simulink model "ESSSimulation_NCR"  (R2025a)
settings: Solver=VariableStepAuto  StartTime=0.0  StopTime=1800  RelTol=1e-3
undefined symbols (not defined in the file or in its folder): battery_builder_rtmsupport, gcbh
libraries: NCR18650BD_98S45P_Library_lib x14, fl_lib x4, nesl_utility x4, simulink x1, SignalEditorBlockLib x1
(part 2 of 2)

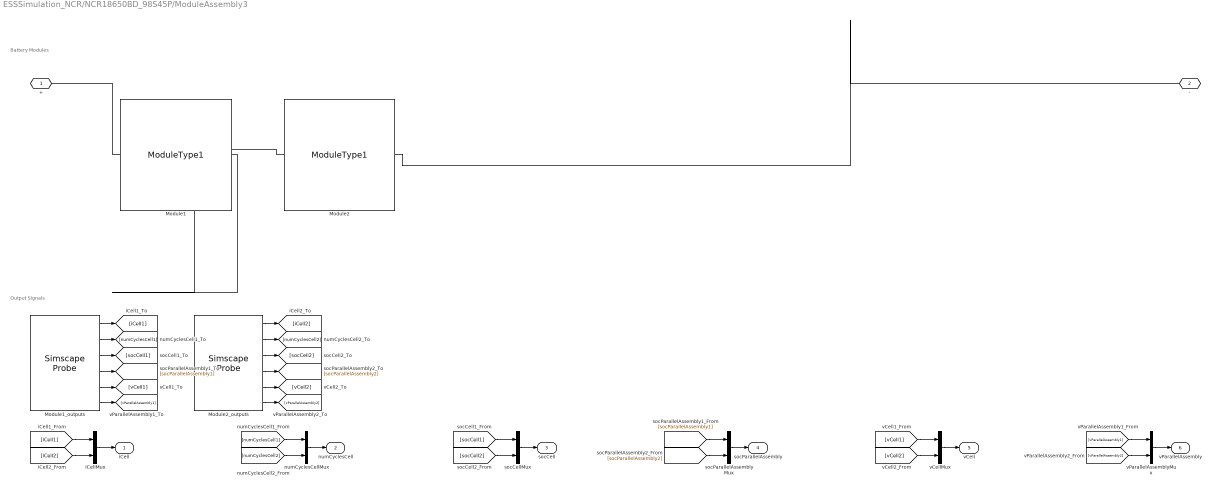
== system ESSSimulation_NCR/NCR18650BD_98S45P/ModuleAssembly3 ==
  note: Battery Modules
  note: Output Signals
  Module1 : NCR18650BD_98S45P_Library_lib/Modules/ModuleType1  SOC_vecCell=[0 0.01 0.02 0.03 0.04 0.05 0.06 0.07 0.08 0.09 0.1 0.11 0.12 0.13 0.14 0.15 0.16 0.17 0.18 0.19 0.2 0.21 0.22 0.23 0.24 0.25 0.26 0.27 0.28 0.29 0.3 0.31 0.32 0.33 0.34 0.35 0.36 0.37 0.38 0.39 0.4 0.41 0.42 0.43 0.44 0.45 0.46 0.47 0.48 0.49 0.5 0.51 0.52 0.53 0.54 0.55 0.56 0.57 0.58 0.59 0.6 0.61 0.62 0.63 0.64 0.65 0.66 0.67 0.68 0.69 0.7 0.71 0.72 0.73 0.74 0.75 0.76 0.77 0.78 0.79 0.8 0.81 0.82 0.83 0.84 0.85 0.86 0.87 0.88 0.89 0.9 0.91 0.92 0.93 0.94 0.95 0.96 0.97 0.98 0.99 1]  V0_vecCell=[2.90003 2.94341 2.98679 3.04987 3.09433 3.12791 3.16031 3.20369 3.23862 3.26689 3.29115 3.31383 3.33202 3.35112 3.36833 3.38413 3.39973 3.41137 3.42149 3.43136 3.44073 3.45027 3.46068 3.47113 3.47814 3.48494 3.49199 3.49905 3.50562 3.51187 3.51861 3.52535 3.53209 3.53818 3.54353 3.54849 3.55353 3.55855 3.56357 3.56831 3.57308 3.57787 3.58264 3.58755 3.5925 3.5985 3.60496 3.61149 3.61805 3.6246 3.63116 3.63855 3.64609 3.65336 3.66064 3.66791 3.67613 3.68522 3.69443 3.70367 3.713 3.72241 3.73154 3.74037 3.7492 3.75786 3.76617 3.77556 3.78485 3.79413 3.8034 3.81149 3.81977 3.82804 3.83631 3.84472 3.85317 3.86155 3.86993 3.87831 3.88686 3.89534 3.90461 3.91454 3.92565 3.93721 3.94924 3.96155 3.97383 3.98598 3.99856 4.01117 4.02361 4.03609 4.04694 4.05695 4.06641 4.07551 4.08514 4.09447 4.10453] V  V_rangeCell=[2.25 Inf] V  R0_vecCell=[0.1741 0.15823 0.14313 0.13285 0.12044 0.10641 0.09605 0.09162 0.08758 0.08349 0.08021 0.07738 0.07487 0.07338 0.07189 0.07117 0.0704 0.06898 0.06755 0.06631 0.06509 0.06388 0.06326 0.06281 0.06182 0.06095 0.06025 0.05955 0.05877 0.05807 0.05761 0.05714 0.05668 0.05611 0.05546 0.0549 0.05439 0.05388 0.05337 0.0528 0.05223 0.05165 0.05106 0.05046 0.04986 0.04945 0.04913 0.04883 0.04854 0.04826 0.04797 0.04782 0.04765 0.0473 0.04695 0.04661 0.04638 0.0463 0.04625 0.04621 0.04624 0.04628 0.04628 0.04623 0.04617 0.04599 0.04573 0.0457 0.04568 0.04565 0.04563 0.04535 0.0451 0.04486 0.04461 0.04446 0.04435 0.04423 0.04411 0.044 0.04372 0.04339 0.04323 0.0432 0.04344 0.04374 0.0441 0.04452 0.04494 0.0454 0.04594 0.0463 0.04649 0.04668 0.04629 0.04541 0.04438 0.04326 0.04154 0.03869 0.03326] Ohm  AHCell=3.153 hr*A  extrapolation_optionCell=simscape.enum.extrapolation.nearest  P=45  S=7  iCell_specify=off  iCell_priority=None  iCell=0 A  iCell_nominal_specify=off  iCell_nominal_value=1  iCell_nominal_unit=A  vCell_specify=off  vCell_priority=None  vCell=0 V  vCell_nominal_specify=off  vCell_nominal_value=1  vCell_nominal_unit=V  socCell_specify=off  socCell_priority=High  socCell=1  socCell_nominal_specify=off  socCell_nominal_value=1  socCell_nominal_unit=1  numCyclesCell_specify=off  numCyclesCell_priority=High  numCyclesCell=0  numCyclesCell_nominal_specify=off  numCyclesCell_nominal_value=1  numCyclesCell_nominal_unit=1  vParallelAssembly_specify=off  vParallelAssembly_priority=None  vParallelAssembly=repmat(0, 7, 1) V  vParallelAssembly_nominal_specify=off  vParallelAssembly_nominal_value=1  vParallelAssembly_nominal_unit=V  socParallelAssembly_specify=off  socParallelAssembly_priority=None  socParallelAssembly=repmat(1, 7, 1)  socParallelAssembly_nominal_specify=off  socParallelAssembly_nominal_value=1  socParallelAssembly_nominal_unit=1
      settings: InternalSimscapePortConfiguration="{\"Bottom\":[{\"id\":\"n\",\"label\":\"-\",\"type\":\"foundation.electrical.electrical\"}],\"Left\":[],\"Right\":[],\"Top\":[{\"id\":\"p\",\"label\":\"+\",\"type\":\"foundation.electrical.electrical\"}]}"
  Module1_outputs : SimscapeProbe  BoundBlock=690  Variables="{\"iCell\":{\"Probing\":\"ON\"},\"numCyclesCell\":{\"Probing\":\"ON\"},\"socCell\":{\"Probing\":\"ON\"},\"socParallelAssembly\":{\"Probing\":\"ON\"},\"vCell\":{\"Probing\":\"ON\"},\"vParallelAssembly\":{\"Probing\":\"ON\"}}"
  Module2 : NCR18650BD_98S45P_Library_lib/Modules/ModuleType1  SOC_vecCell=[0 0.01 0.02 0.03 0.04 0.05 0.06 0.07 0.08 0.09 0.1 0.11 0.12 0.13 0.14 0.15 0.16 0.17 0.18 0.19 0.2 0.21 0.22 0.23 0.24 0.25 0.26 0.27 0.28 0.29 0.3 0.31 0.32 0.33 0.34 0.35 0.36 0.37 0.38 0.39 0.4 0.41 0.42 0.43 0.44 0.45 0.46 0.47 0.48 0.49 0.5 0.51 0.52 0.53 0.54 0.55 0.56 0.57 0.58 0.59 0.6 0.61 0.62 0.63 0.64 0.65 0.66 0.67 0.68 0.69 0.7 0.71 0.72 0.73 0.74 0.75 0.76 0.77 0.78 0.79 0.8 0.81 0.82 0.83 0.84 0.85 0.86 0.87 0.88 0.89 0.9 0.91 0.92 0.93 0.94 0.95 0.96 0.97 0.98 0.99 1]  V0_vecCell=[2.90003 2.94341 2.98679 3.04987 3.09433 3.12791 3.16031 3.20369 3.23862 3.26689 3.29115 3.31383 3.33202 3.35112 3.36833 3.38413 3.39973 3.41137 3.42149 3.43136 3.44073 3.45027 3.46068 3.47113 3.47814 3.48494 3.49199 3.49905 3.50562 3.51187 3.51861 3.52535 3.53209 3.53818 3.54353 3.54849 3.55353 3.55855 3.56357 3.56831 3.57308 3.57787 3.58264 3.58755 3.5925 3.5985 3.60496 3.61149 3.61805 3.6246 3.63116 3.63855 3.64609 3.65336 3.66064 3.66791 3.67613 3.68522 3.69443 3.70367 3.713 3.72241 3.73154 3.74037 3.7492 3.75786 3.76617 3.77556 3.78485 3.79413 3.8034 3.81149 3.81977 3.82804 3.83631 3.84472 3.85317 3.86155 3.86993 3.87831 3.88686 3.89534 3.90461 3.91454 3.92565 3.93721 3.94924 3.96155 3.97383 3.98598 3.99856 4.01117 4.02361 4.03609 4.04694 4.05695 4.06641 4.07551 4.08514 4.09447 4.10453] V  V_rangeCell=[2.25 Inf] V  R0_vecCell=[0.1741 0.15823 0.14313 0.13285 0.12044 0.10641 0.09605 0.09162 0.08758 0.08349 0.08021 0.07738 0.07487 0.07338 0.07189 0.07117 0.0704 0.06898 0.06755 0.06631 0.06509 0.06388 0.06326 0.06281 0.06182 0.06095 0.06025 0.05955 0.05877 0.05807 0.05761 0.05714 0.05668 0.05611 0.05546 0.0549 0.05439 0.05388 0.05337 0.0528 0.05223 0.05165 0.05106 0.05046 0.04986 0.04945 0.04913 0.04883 0.04854 0.04826 0.04797 0.04782 0.04765 0.0473 0.04695 0.04661 0.04638 0.0463 0.04625 0.04621 0.04624 0.04628 0.04628 0.04623 0.04617 0.04599 0.04573 0.0457 0.04568 0.04565 0.04563 0.04535 0.0451 0.04486 0.04461 0.04446 0.04435 0.04423 0.04411 0.044 0.04372 0.04339 0.04323 0.0432 0.04344 0.04374 0.0441 0.04452 0.04494 0.0454 0.04594 0.0463 0.04649 0.04668 0.04629 0.04541 0.04438 0.04326 0.04154 0.03869 0.03326] Ohm  AHCell=3.153 hr*A  extrapolation_optionCell=simscape.enum.extrapolation.nearest  P=45  S=7  iCell_specify=off  iCell_priority=None  iCell=0 A  iCell_nominal_specify=off  iCell_nominal_value=1  iCell_nominal_unit=A  vCell_specify=off  vCell_priority=None  vCell=0 V  vCell_nominal_specify=off  vCell_nominal_value=1  vCell_nominal_unit=V  socCell_specify=off  socCell_priority=High  socCell=1  socCell_nominal_specify=off  socCell_nominal_value=1  socCell_nominal_unit=1  numCyclesCell_specify=off  numCyclesCell_priority=High  numCyclesCell=0  numCyclesCell_nominal_specify=off  numCyclesCell_nominal_value=1  numCyclesCell_nominal_unit=1  vParallelAssembly_specify=off  vParallelAssembly_priority=None  vParallelAssembly=repmat(0, 7, 1) V  vParallelAssembly_nominal_specify=off  vParallelAssembly_nominal_value=1  vParallelAssembly_nominal_unit=V  socParallelAssembly_specify=off  socParallelAssembly_priority=None  socParallelAssembly=repmat(1, 7, 1)  socParallelAssembly_nominal_specify=off  socParallelAssembly_nominal_value=1  socParallelAssembly_nominal_unit=1
      settings: InternalSimscapePortConfiguration="{\"Bottom\":[{\"id\":\"n\",\"label\":\"-\",\"type\":\"foundation.electrical.electrical\"}],\"Left\":[],\"Right\":[],\"Top\":[{\"id\":\"p\",\"label\":\"+\",\"type\":\"foundation.electrical.electrical\"}]}"
  Module2_outputs : SimscapeProbe  BoundBlock=692  Variables="{\"iCell\":{\"Probing\":\"ON\"},\"numCyclesCell\":{\"Probing\":\"ON\"},\"socCell\":{\"Probing\":\"ON\"},\"socParallelAssembly\":{\"Probing\":\"ON\"},\"vCell\":{\"Probing\":\"ON\"},\"vParallelAssembly\":{\"Probing\":\"ON\"}}"
  iCellMux : Mux  Inputs=2
  numCyclesCellMux : Mux  Inputs=2
  socCellMux : Mux  Inputs=2
  socParallelAssemblyMux : Mux  Inputs=2
  vCellMux : Mux  Inputs=2
  vParallelAssemblyMux : Mux  Inputs=2
  + : PMIOPort  Side=Left
  - : PMIOPort  Port=2  Side=Right
  iCell : Outport
  numCyclesCell : Outport  Port=2
  socCell : Outport  Port=3
  socParallelAssembly : Outport  Port=4
  vCell : Outport  Port=5
  vParallelAssembly : Outport  Port=6
  wires:
  Module1_outputs/1 -> [iCell1]
  iCellMux/1 -> iCell/1
  [iCell1] -> iCellMux/1
  Module1_outputs/2 -> [numCyclesCell1]
  numCyclesCellMux/1 -> numCyclesCell/1
  [numCyclesCell1] -> numCyclesCellMux/1
  Module1_outputs/3 -> [socCell1]
  socCellMux/1 -> socCell/1
  [socCell1] -> socCellMux/1
  Module1_outputs/4 -> [socParallelAssembly1]
  socParallelAssemblyMux/1 -> socParallelAssembly/1
  [socParallelAssembly1] -> socParallelAssemblyMux/1
  Module1_outputs/5 -> [vCell1]
  vCellMux/1 -> vCell/1
  [vCell1] -> vCellMux/1
  Module1_outputs/6 -> [vParallelAssembly1]
  vParallelAssemblyMux/1 -> vParallelAssembly/1
  [vParallelAssembly1] -> vParallelAssemblyMux/1
  Module2_outputs/1 -> [iCell2]
  [iCell2] -> iCellMux/2
  Module2_outputs/2 -> [numCyclesCell2]
  [numCyclesCell2] -> numCyclesCellMux/2
  Module2_outputs/3 -> [socCell2]
  [socCell2] -> socCellMux/2
  Module2_outputs/4 -> [socParallelAssembly2]
  [socParallelAssembly2] -> socParallelAssemblyMux/2
  Module2_outputs/5 -> [vCell2]
  [vCell2] -> vCellMux/2
  Module2_outputs/6 -> [vParallelAssembly2]
  [vParallelAssembly2] -> vParallelAssemblyMux/2
  connections:
  Module2/LConn1 -- Module1/RConn1
  Module1/LConn1 -- +/RConn1
  Module2/RConn1 -- -/RConn1

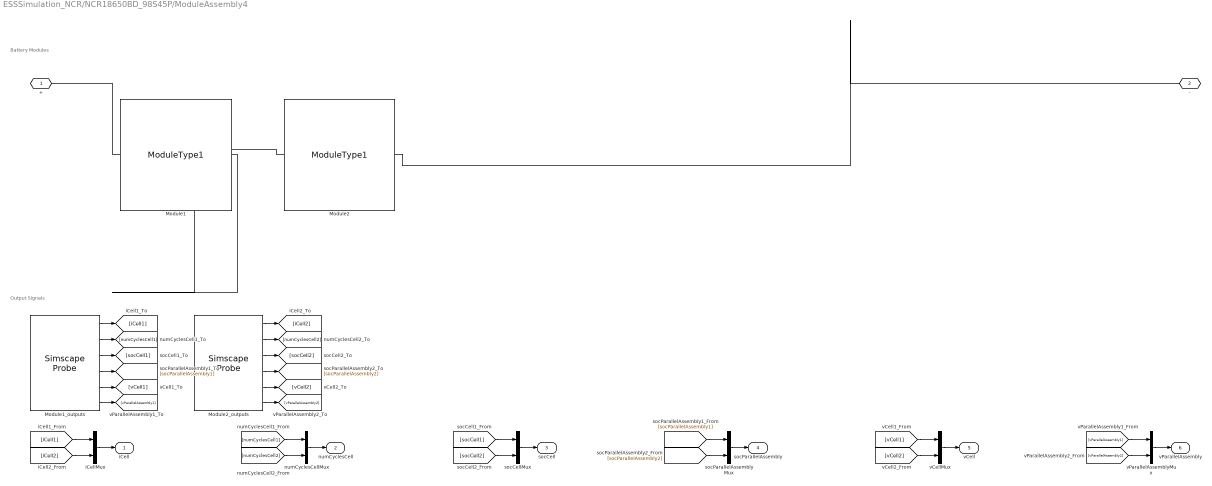
== system ESSSimulation_NCR/NCR18650BD_98S45P/ModuleAssembly4 ==
  note: Battery Modules
  note: Output Signals
  Module1 : NCR18650BD_98S45P_Library_lib/Modules/ModuleType1  SOC_vecCell=[0 0.01 0.02 0.03 0.04 0.05 0.06 0.07 0.08 0.09 0.1 0.11 0.12 0.13 0.14 0.15 0.16 0.17 0.18 0.19 0.2 0.21 0.22 0.23 0.24 0.25 0.26 0.27 0.28 0.29 0.3 0.31 0.32 0.33 0.34 0.35 0.36 0.37 0.38 0.39 0.4 0.41 0.42 0.43 0.44 0.45 0.46 0.47 0.48 0.49 0.5 0.51 0.52 0.53 0.54 0.55 0.56 0.57 0.58 0.59 0.6 0.61 0.62 0.63 0.64 0.65 0.66 0.67 0.68 0.69 0.7 0.71 0.72 0.73 0.74 0.75 0.76 0.77 0.78 0.79 0.8 0.81 0.82 0.83 0.84 0.85 0.86 0.87 0.88 0.89 0.9 0.91 0.92 0.93 0.94 0.95 0.96 0.97 0.98 0.99 1]  V0_vecCell=[2.90003 2.94341 2.98679 3.04987 3.09433 3.12791 3.16031 3.20369 3.23862 3.26689 3.29115 3.31383 3.33202 3.35112 3.36833 3.38413 3.39973 3.41137 3.42149 3.43136 3.44073 3.45027 3.46068 3.47113 3.47814 3.48494 3.49199 3.49905 3.50562 3.51187 3.51861 3.52535 3.53209 3.53818 3.54353 3.54849 3.55353 3.55855 3.56357 3.56831 3.57308 3.57787 3.58264 3.58755 3.5925 3.5985 3.60496 3.61149 3.61805 3.6246 3.63116 3.63855 3.64609 3.65336 3.66064 3.66791 3.67613 3.68522 3.69443 3.70367 3.713 3.72241 3.73154 3.74037 3.7492 3.75786 3.76617 3.77556 3.78485 3.79413 3.8034 3.81149 3.81977 3.82804 3.83631 3.84472 3.85317 3.86155 3.86993 3.87831 3.88686 3.89534 3.90461 3.91454 3.92565 3.93721 3.94924 3.96155 3.97383 3.98598 3.99856 4.01117 4.02361 4.03609 4.04694 4.05695 4.06641 4.07551 4.08514 4.09447 4.10453] V  V_rangeCell=[2.25 Inf] V  R0_vecCell=[0.1741 0.15823 0.14313 0.13285 0.12044 0.10641 0.09605 0.09162 0.08758 0.08349 0.08021 0.07738 0.07487 0.07338 0.07189 0.07117 0.0704 0.06898 0.06755 0.06631 0.06509 0.06388 0.06326 0.06281 0.06182 0.06095 0.06025 0.05955 0.05877 0.05807 0.05761 0.05714 0.05668 0.05611 0.05546 0.0549 0.05439 0.05388 0.05337 0.0528 0.05223 0.05165 0.05106 0.05046 0.04986 0.04945 0.04913 0.04883 0.04854 0.04826 0.04797 0.04782 0.04765 0.0473 0.04695 0.04661 0.04638 0.0463 0.04625 0.04621 0.04624 0.04628 0.04628 0.04623 0.04617 0.04599 0.04573 0.0457 0.04568 0.04565 0.04563 0.04535 0.0451 0.04486 0.04461 0.04446 0.04435 0.04423 0.04411 0.044 0.04372 0.04339 0.04323 0.0432 0.04344 0.04374 0.0441 0.04452 0.04494 0.0454 0.04594 0.0463 0.04649 0.04668 0.04629 0.04541 0.04438 0.04326 0.04154 0.03869 0.03326] Ohm  AHCell=3.153 hr*A  extrapolation_optionCell=simscape.enum.extrapolation.nearest  P=45  S=7  iCell_specify=off  iCell_priority=None  iCell=0 A  iCell_nominal_specify=off  iCell_nominal_value=1  iCell_nominal_unit=A  vCell_specify=off  vCell_priority=None  vCell=0 V  vCell_nominal_specify=off  vCell_nominal_value=1  vCell_nominal_unit=V  socCell_specify=off  socCell_priority=High  socCell=1  socCell_nominal_specify=off  socCell_nominal_value=1  socCell_nominal_unit=1  numCyclesCell_specify=off  numCyclesCell_priority=High  numCyclesCell=0  numCyclesCell_nominal_specify=off  numCyclesCell_nominal_value=1  numCyclesCell_nominal_unit=1  vParallelAssembly_specify=off  vParallelAssembly_priority=None  vParallelAssembly=repmat(0, 7, 1) V  vParallelAssembly_nominal_specify=off  vParallelAssembly_nominal_value=1  vParallelAssembly_nominal_unit=V  socParallelAssembly_specify=off  socParallelAssembly_priority=None  socParallelAssembly=repmat(1, 7, 1)  socParallelAssembly_nominal_specify=off  socParallelAssembly_nominal_value=1  socParallelAssembly_nominal_unit=1
      settings: InternalSimscapePortConfiguration="{\"Bottom\":[{\"id\":\"n\",\"label\":\"-\",\"type\":\"foundation.electrical.electrical\"}],\"Left\":[],\"Right\":[],\"Top\":[{\"id\":\"p\",\"label\":\"+\",\"type\":\"foundation.electrical.electrical\"}]}"
  Module1_outputs : SimscapeProbe  BoundBlock=735  Variables="{\"iCell\":{\"Probing\":\"ON\"},\"numCyclesCell\":{\"Probing\":\"ON\"},\"socCell\":{\"Probing\":\"ON\"},\"socParallelAssembly\":{\"Probing\":\"ON\"},\"vCell\":{\"Probing\":\"ON\"},\"vParallelAssembly\":{\"Probing\":\"ON\"}}"
  Module2 : NCR18650BD_98S45P_Library_lib/Modules/ModuleType1  SOC_vecCell=[0 0.01 0.02 0.03 0.04 0.05 0.06 0.07 0.08 0.09 0.1 0.11 0.12 0.13 0.14 0.15 0.16 0.17 0.18 0.19 0.2 0.21 0.22 0.23 0.24 0.25 0.26 0.27 0.28 0.29 0.3 0.31 0.32 0.33 0.34 0.35 0.36 0.37 0.38 0.39 0.4 0.41 0.42 0.43 0.44 0.45 0.46 0.47 0.48 0.49 0.5 0.51 0.52 0.53 0.54 0.55 0.56 0.57 0.58 0.59 0.6 0.61 0.62 0.63 0.64 0.65 0.66 0.67 0.68 0.69 0.7 0.71 0.72 0.73 0.74 0.75 0.76 0.77 0.78 0.79 0.8 0.81 0.82 0.83 0.84 0.85 0.86 0.87 0.88 0.89 0.9 0.91 0.92 0.93 0.94 0.95 0.96 0.97 0.98 0.99 1]  V0_vecCell=[2.90003 2.94341 2.98679 3.04987 3.09433 3.12791 3.16031 3.20369 3.23862 3.26689 3.29115 3.31383 3.33202 3.35112 3.36833 3.38413 3.39973 3.41137 3.42149 3.43136 3.44073 3.45027 3.46068 3.47113 3.47814 3.48494 3.49199 3.49905 3.50562 3.51187 3.51861 3.52535 3.53209 3.53818 3.54353 3.54849 3.55353 3.55855 3.56357 3.56831 3.57308 3.57787 3.58264 3.58755 3.5925 3.5985 3.60496 3.61149 3.61805 3.6246 3.63116 3.63855 3.64609 3.65336 3.66064 3.66791 3.67613 3.68522 3.69443 3.70367 3.713 3.72241 3.73154 3.74037 3.7492 3.75786 3.76617 3.77556 3.78485 3.79413 3.8034 3.81149 3.81977 3.82804 3.83631 3.84472 3.85317 3.86155 3.86993 3.87831 3.88686 3.89534 3.90461 3.91454 3.92565 3.93721 3.94924 3.96155 3.97383 3.98598 3.99856 4.01117 4.02361 4.03609 4.04694 4.05695 4.06641 4.07551 4.08514 4.09447 4.10453] V  V_rangeCell=[2.25 Inf] V  R0_vecCell=[0.1741 0.15823 0.14313 0.13285 0.12044 0.10641 0.09605 0.09162 0.08758 0.08349 0.08021 0.07738 0.07487 0.07338 0.07189 0.07117 0.0704 0.06898 0.06755 0.06631 0.06509 0.06388 0.06326 0.06281 0.06182 0.06095 0.06025 0.05955 0.05877 0.05807 0.05761 0.05714 0.05668 0.05611 0.05546 0.0549 0.05439 0.05388 0.05337 0.0528 0.05223 0.05165 0.05106 0.05046 0.04986 0.04945 0.04913 0.04883 0.04854 0.04826 0.04797 0.04782 0.04765 0.0473 0.04695 0.04661 0.04638 0.0463 0.04625 0.04621 0.04624 0.04628 0.04628 0.04623 0.04617 0.04599 0.04573 0.0457 0.04568 0.04565 0.04563 0.04535 0.0451 0.04486 0.04461 0.04446 0.04435 0.04423 0.04411 0.044 0.04372 0.04339 0.04323 0.0432 0.04344 0.04374 0.0441 0.04452 0.04494 0.0454 0.04594 0.0463 0.04649 0.04668 0.04629 0.04541 0.04438 0.04326 0.04154 0.03869 0.03326] Ohm  AHCell=3.153 hr*A  extrapolation_optionCell=simscape.enum.extrapolation.nearest  P=45  S=7  iCell_specify=off  iCell_priority=None  iCell=0 A  iCell_nominal_specify=off  iCell_nominal_value=1  iCell_nominal_unit=A  vCell_specify=off  vCell_priority=None  vCell=0 V  vCell_nominal_specify=off  vCell_nominal_value=1  vCell_nominal_unit=V  socCell_specify=off  socCell_priority=High  socCell=1  socCell_nominal_specify=off  socCell_nominal_value=1  socCell_nominal_unit=1  numCyclesCell_specify=off  numCyclesCell_priority=High  numCyclesCell=0  numCyclesCell_nominal_specify=off  numCyclesCell_nominal_value=1  numCyclesCell_nominal_unit=1  vParallelAssembly_specify=off  vParallelAssembly_priority=None  vParallelAssembly=repmat(0, 7, 1) V  vParallelAssembly_nominal_specify=off  vParallelAssembly_nominal_value=1  vParallelAssembly_nominal_unit=V  socParallelAssembly_specify=off  socParallelAssembly_priority=None  socParallelAssembly=repmat(1, 7, 1)  socParallelAssembly_nominal_specify=off  socParallelAssembly_nominal_value=1  socParallelAssembly_nominal_unit=1
      settings: InternalSimscapePortConfiguration="{\"Bottom\":[{\"id\":\"n\",\"label\":\"-\",\"type\":\"foundation.electrical.electrical\"}],\"Left\":[],\"Right\":[],\"Top\":[{\"id\":\"p\",\"label\":\"+\",\"type\":\"foundation.electrical.electrical\"}]}"
  Module2_outputs : SimscapeProbe  BoundBlock=737  Variables="{\"iCell\":{\"Probing\":\"ON\"},\"numCyclesCell\":{\"Probing\":\"ON\"},\"socCell\":{\"Probing\":\"ON\"},\"socParallelAssembly\":{\"Probing\":\"ON\"},\"vCell\":{\"Probing\":\"ON\"},\"vParallelAssembly\":{\"Probing\":\"ON\"}}"
  iCellMux : Mux  Inputs=2
  numCyclesCellMux : Mux  Inputs=2
  socCellMux : Mux  Inputs=2
  socParallelAssemblyMux : Mux  Inputs=2
  vCellMux : Mux  Inputs=2
  vParallelAssemblyMux : Mux  Inputs=2
  + : PMIOPort  Side=Left
  - : PMIOPort  Port=2  Side=Right
  iCell : Outport
  numCyclesCell : Outport  Port=2
  socCell : Outport  Port=3
  socParallelAssembly : Outport  Port=4
  vCell : Outport  Port=5
  vParallelAssembly : Outport  Port=6
  wires:
  Module1_outputs/1 -> [iCell1]
  iCellMux/1 -> iCell/1
  [iCell1] -> iCellMux/1
  Module1_outputs/2 -> [numCyclesCell1]
  numCyclesCellMux/1 -> numCyclesCell/1
  [numCyclesCell1] -> numCyclesCellMux/1
  Module1_outputs/3 -> [socCell1]
  socCellMux/1 -> socCell/1
  [socCell1] -> socCellMux/1
  Module1_outputs/4 -> [socParallelAssembly1]
  socParallelAssemblyMux/1 -> socParallelAssembly/1
  [socParallelAssembly1] -> socParallelAssemblyMux/1
  Module1_outputs/5 -> [vCell1]
  vCellMux/1 -> vCell/1
  [vCell1] -> vCellMux/1
  Module1_outputs/6 -> [vParallelAssembly1]
  vParallelAssemblyMux/1 -> vParallelAssembly/1
  [vParallelAssembly1] -> vParallelAssemblyMux/1
  Module2_outputs/1 -> [iCell2]
  [iCell2] -> iCellMux/2
  Module2_outputs/2 -> [numCyclesCell2]
  [numCyclesCell2] -> numCyclesCellMux/2
  Module2_outputs/3 -> [socCell2]
  [socCell2] -> socCellMux/2
  Module2_outputs/4 -> [socParallelAssembly2]
  [socParallelAssembly2] -> socParallelAssemblyMux/2
  Module2_outputs/5 -> [vCell2]
  [vCell2] -> vCellMux/2
  Module2_outputs/6 -> [vParallelAssembly2]
  [vParallelAssembly2] -> vParallelAssemblyMux/2
  connections:
  Module2/LConn1 -- Module1/RConn1
  Module1/LConn1 -- +/RConn1
  Module2/RConn1 -- -/RConn1

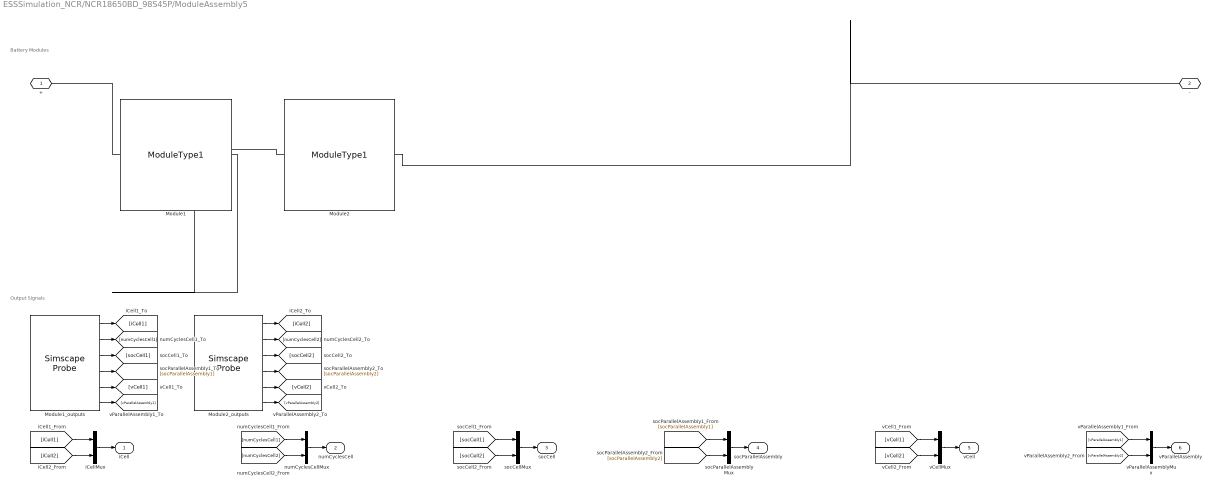
== system ESSSimulation_NCR/NCR18650BD_98S45P/ModuleAssembly5 ==
  note: Battery Modules
  note: Output Signals
  Module1 : NCR18650BD_98S45P_Library_lib/Modules/ModuleType1  SOC_vecCell=[0 0.01 0.02 0.03 0.04 0.05 0.06 0.07 0.08 0.09 0.1 0.11 0.12 0.13 0.14 0.15 0.16 0.17 0.18 0.19 0.2 0.21 0.22 0.23 0.24 0.25 0.26 0.27 0.28 0.29 0.3 0.31 0.32 0.33 0.34 0.35 0.36 0.37 0.38 0.39 0.4 0.41 0.42 0.43 0.44 0.45 0.46 0.47 0.48 0.49 0.5 0.51 0.52 0.53 0.54 0.55 0.56 0.57 0.58 0.59 0.6 0.61 0.62 0.63 0.64 0.65 0.66 0.67 0.68 0.69 0.7 0.71 0.72 0.73 0.74 0.75 0.76 0.77 0.78 0.79 0.8 0.81 0.82 0.83 0.84 0.85 0.86 0.87 0.88 0.89 0.9 0.91 0.92 0.93 0.94 0.95 0.96 0.97 0.98 0.99 1]  V0_vecCell=[2.90003 2.94341 2.98679 3.04987 3.09433 3.12791 3.16031 3.20369 3.23862 3.26689 3.29115 3.31383 3.33202 3.35112 3.36833 3.38413 3.39973 3.41137 3.42149 3.43136 3.44073 3.45027 3.46068 3.47113 3.47814 3.48494 3.49199 3.49905 3.50562 3.51187 3.51861 3.52535 3.53209 3.53818 3.54353 3.54849 3.55353 3.55855 3.56357 3.56831 3.57308 3.57787 3.58264 3.58755 3.5925 3.5985 3.60496 3.61149 3.61805 3.6246 3.63116 3.63855 3.64609 3.65336 3.66064 3.66791 3.67613 3.68522 3.69443 3.70367 3.713 3.72241 3.73154 3.74037 3.7492 3.75786 3.76617 3.77556 3.78485 3.79413 3.8034 3.81149 3.81977 3.82804 3.83631 3.84472 3.85317 3.86155 3.86993 3.87831 3.88686 3.89534 3.90461 3.91454 3.92565 3.93721 3.94924 3.96155 3.97383 3.98598 3.99856 4.01117 4.02361 4.03609 4.04694 4.05695 4.06641 4.07551 4.08514 4.09447 4.10453] V  V_rangeCell=[2.25 Inf] V  R0_vecCell=[0.1741 0.15823 0.14313 0.13285 0.12044 0.10641 0.09605 0.09162 0.08758 0.08349 0.08021 0.07738 0.07487 0.07338 0.07189 0.07117 0.0704 0.06898 0.06755 0.06631 0.06509 0.06388 0.06326 0.06281 0.06182 0.06095 0.06025 0.05955 0.05877 0.05807 0.05761 0.05714 0.05668 0.05611 0.05546 0.0549 0.05439 0.05388 0.05337 0.0528 0.05223 0.05165 0.05106 0.05046 0.04986 0.04945 0.04913 0.04883 0.04854 0.04826 0.04797 0.04782 0.04765 0.0473 0.04695 0.04661 0.04638 0.0463 0.04625 0.04621 0.04624 0.04628 0.04628 0.04623 0.04617 0.04599 0.04573 0.0457 0.04568 0.04565 0.04563 0.04535 0.0451 0.04486 0.04461 0.04446 0.04435 0.04423 0.04411 0.044 0.04372 0.04339 0.04323 0.0432 0.04344 0.04374 0.0441 0.04452 0.04494 0.0454 0.04594 0.0463 0.04649 0.04668 0.04629 0.04541 0.04438 0.04326 0.04154 0.03869 0.03326] Ohm  AHCell=3.153 hr*A  extrapolation_optionCell=simscape.enum.extrapolation.nearest  P=45  S=7  iCell_specify=off  iCell_priority=None  iCell=0 A  iCell_nominal_specify=off  iCell_nominal_value=1  iCell_nominal_unit=A  vCell_specify=off  vCell_priority=None  vCell=0 V  vCell_nominal_specify=off  vCell_nominal_value=1  vCell_nominal_unit=V  socCell_specify=off  socCell_priority=High  socCell=1  socCell_nominal_specify=off  socCell_nominal_value=1  socCell_nominal_unit=1  numCyclesCell_specify=off  numCyclesCell_priority=High  numCyclesCell=0  numCyclesCell_nominal_specify=off  numCyclesCell_nominal_value=1  numCyclesCell_nominal_unit=1  vParallelAssembly_specify=off  vParallelAssembly_priority=None  vParallelAssembly=repmat(0, 7, 1) V  vParallelAssembly_nominal_specify=off  vParallelAssembly_nominal_value=1  vParallelAssembly_nominal_unit=V  socParallelAssembly_specify=off  socParallelAssembly_priority=None  socParallelAssembly=repmat(1, 7, 1)  socParallelAssembly_nominal_specify=off  socParallelAssembly_nominal_value=1  socParallelAssembly_nominal_unit=1
      settings: InternalSimscapePortConfiguration="{\"Bottom\":[{\"id\":\"n\",\"label\":\"-\",\"type\":\"foundation.electrical.electrical\"}],\"Left\":[],\"Right\":[],\"Top\":[{\"id\":\"p\",\"label\":\"+\",\"type\":\"foundation.electrical.electrical\"}]}"
  Module1_outputs : SimscapeProbe  BoundBlock=780  Variables="{\"iCell\":{\"Probing\":\"ON\"},\"numCyclesCell\":{\"Probing\":\"ON\"},\"socCell\":{\"Probing\":\"ON\"},\"socParallelAssembly\":{\"Probing\":\"ON\"},\"vCell\":{\"Probing\":\"ON\"},\"vParallelAssembly\":{\"Probing\":\"ON\"}}"
  Module2 : NCR18650BD_98S45P_Library_lib/Modules/ModuleType1  SOC_vecCell=[0 0.01 0.02 0.03 0.04 0.05 0.06 0.07 0.08 0.09 0.1 0.11 0.12 0.13 0.14 0.15 0.16 0.17 0.18 0.19 0.2 0.21 0.22 0.23 0.24 0.25 0.26 0.27 0.28 0.29 0.3 0.31 0.32 0.33 0.34 0.35 0.36 0.37 0.38 0.39 0.4 0.41 0.42 0.43 0.44 0.45 0.46 0.47 0.48 0.49 0.5 0.51 0.52 0.53 0.54 0.55 0.56 0.57 0.58 0.59 0.6 0.61 0.62 0.63 0.64 0.65 0.66 0.67 0.68 0.69 0.7 0.71 0.72 0.73 0.74 0.75 0.76 0.77 0.78 0.79 0.8 0.81 0.82 0.83 0.84 0.85 0.86 0.87 0.88 0.89 0.9 0.91 0.92 0.93 0.94 0.95 0.96 0.97 0.98 0.99 1]  V0_vecCell=[2.90003 2.94341 2.98679 3.04987 3.09433 3.12791 3.16031 3.20369 3.23862 3.26689 3.29115 3.31383 3.33202 3.35112 3.36833 3.38413 3.39973 3.41137 3.42149 3.43136 3.44073 3.45027 3.46068 3.47113 3.47814 3.48494 3.49199 3.49905 3.50562 3.51187 3.51861 3.52535 3.53209 3.53818 3.54353 3.54849 3.55353 3.55855 3.56357 3.56831 3.57308 3.57787 3.58264 3.58755 3.5925 3.5985 3.60496 3.61149 3.61805 3.6246 3.63116 3.63855 3.64609 3.65336 3.66064 3.66791 3.67613 3.68522 3.69443 3.70367 3.713 3.72241 3.73154 3.74037 3.7492 3.75786 3.76617 3.77556 3.78485 3.79413 3.8034 3.81149 3.81977 3.82804 3.83631 3.84472 3.85317 3.86155 3.86993 3.87831 3.88686 3.89534 3.90461 3.91454 3.92565 3.93721 3.94924 3.96155 3.97383 3.98598 3.99856 4.01117 4.02361 4.03609 4.04694 4.05695 4.06641 4.07551 4.08514 4.09447 4.10453] V  V_rangeCell=[2.25 Inf] V  R0_vecCell=[0.1741 0.15823 0.14313 0.13285 0.12044 0.10641 0.09605 0.09162 0.08758 0.08349 0.08021 0.07738 0.07487 0.07338 0.07189 0.07117 0.0704 0.06898 0.06755 0.06631 0.06509 0.06388 0.06326 0.06281 0.06182 0.06095 0.06025 0.05955 0.05877 0.05807 0.05761 0.05714 0.05668 0.05611 0.05546 0.0549 0.05439 0.05388 0.05337 0.0528 0.05223 0.05165 0.05106 0.05046 0.04986 0.04945 0.04913 0.04883 0.04854 0.04826 0.04797 0.04782 0.04765 0.0473 0.04695 0.04661 0.04638 0.0463 0.04625 0.04621 0.04624 0.04628 0.04628 0.04623 0.04617 0.04599 0.04573 0.0457 0.04568 0.04565 0.04563 0.04535 0.0451 0.04486 0.04461 0.04446 0.04435 0.04423 0.04411 0.044 0.04372 0.04339 0.04323 0.0432 0.04344 0.04374 0.0441 0.04452 0.04494 0.0454 0.04594 0.0463 0.04649 0.04668 0.04629 0.04541 0.04438 0.04326 0.04154 0.03869 0.03326] Ohm  AHCell=3.153 hr*A  extrapolation_optionCell=simscape.enum.extrapolation.nearest  P=45  S=7  iCell_specify=off  iCell_priority=None  iCell=0 A  iCell_nominal_specify=off  iCell_nominal_value=1  iCell_nominal_unit=A  vCell_specify=off  vCell_priority=None  vCell=0 V  vCell_nominal_specify=off  vCell_nominal_value=1  vCell_nominal_unit=V  socCell_specify=off  socCell_priority=High  socCell=1  socCell_nominal_specify=off  socCell_nominal_value=1  socCell_nominal_unit=1  numCyclesCell_specify=off  numCyclesCell_priority=High  numCyclesCell=0  numCyclesCell_nominal_specify=off  numCyclesCell_nominal_value=1  numCyclesCell_nominal_unit=1  vParallelAssembly_specify=off  vParallelAssembly_priority=None  vParallelAssembly=repmat(0, 7, 1) V  vParallelAssembly_nominal_specify=off  vParallelAssembly_nominal_value=1  vParallelAssembly_nominal_unit=V  socParallelAssembly_specify=off  socParallelAssembly_priority=None  socParallelAssembly=repmat(1, 7, 1)  socParallelAssembly_nominal_specify=off  socParallelAssembly_nominal_value=1  socParallelAssembly_nominal_unit=1
      settings: InternalSimscapePortConfiguration="{\"Bottom\":[{\"id\":\"n\",\"label\":\"-\",\"type\":\"foundation.electrical.electrical\"}],\"Left\":[],\"Right\":[],\"Top\":[{\"id\":\"p\",\"label\":\"+\",\"type\":\"foundation.electrical.electrical\"}]}"
  Module2_outputs : SimscapeProbe  BoundBlock=782  Variables="{\"iCell\":{\"Probing\":\"ON\"},\"numCyclesCell\":{\"Probing\":\"ON\"},\"socCell\":{\"Probing\":\"ON\"},\"socParallelAssembly\":{\"Probing\":\"ON\"},\"vCell\":{\"Probing\":\"ON\"},\"vParallelAssembly\":{\"Probing\":\"ON\"}}"
  iCellMux : Mux  Inputs=2
  numCyclesCellMux : Mux  Inputs=2
  socCellMux : Mux  Inputs=2
  socParallelAssemblyMux : Mux  Inputs=2
  vCellMux : Mux  Inputs=2
  vParallelAssemblyMux : Mux  Inputs=2
  + : PMIOPort  Side=Left
  - : PMIOPort  Port=2  Side=Right
  iCell : Outport
  numCyclesCell : Outport  Port=2
  socCell : Outport  Port=3
  socParallelAssembly : Outport  Port=4
  vCell : Outport  Port=5
  vParallelAssembly : Outport  Port=6
  wires:
  Module1_outputs/1 -> [iCell1]
  iCellMux/1 -> iCell/1
  [iCell1] -> iCellMux/1
  Module1_outputs/2 -> [numCyclesCell1]
  numCyclesCellMux/1 -> numCyclesCell/1
  [numCyclesCell1] -> numCyclesCellMux/1
  Module1_outputs/3 -> [socCell1]
  socCellMux/1 -> socCell/1
  [socCell1] -> socCellMux/1
  Module1_outputs/4 -> [socParallelAssembly1]
  socParallelAssemblyMux/1 -> socParallelAssembly/1
  [socParallelAssembly1] -> socParallelAssemblyMux/1
  Module1_outputs/5 -> [vCell1]
  vCellMux/1 -> vCell/1
  [vCell1] -> vCellMux/1
  Module1_outputs/6 -> [vParallelAssembly1]
  vParallelAssemblyMux/1 -> vParallelAssembly/1
  [vParallelAssembly1] -> vParallelAssemblyMux/1
  Module2_outputs/1 -> [iCell2]
  [iCell2] -> iCellMux/2
  Module2_outputs/2 -> [numCyclesCell2]
  [numCyclesCell2] -> numCyclesCellMux/2
  Module2_outputs/3 -> [socCell2]
  [socCell2] -> socCellMux/2
  Module2_outputs/4 -> [socParallelAssembly2]
  [socParallelAssembly2] -> socParallelAssemblyMux/2
  Module2_outputs/5 -> [vCell2]
  [vCell2] -> vCellMux/2
  Module2_outputs/6 -> [vParallelAssembly2]
  [vParallelAssembly2] -> vParallelAssemblyMux/2
  connections:
  Module2/LConn1 -- Module1/RConn1
  Module1/LConn1 -- +/RConn1
  Module2/RConn1 -- -/RConn1

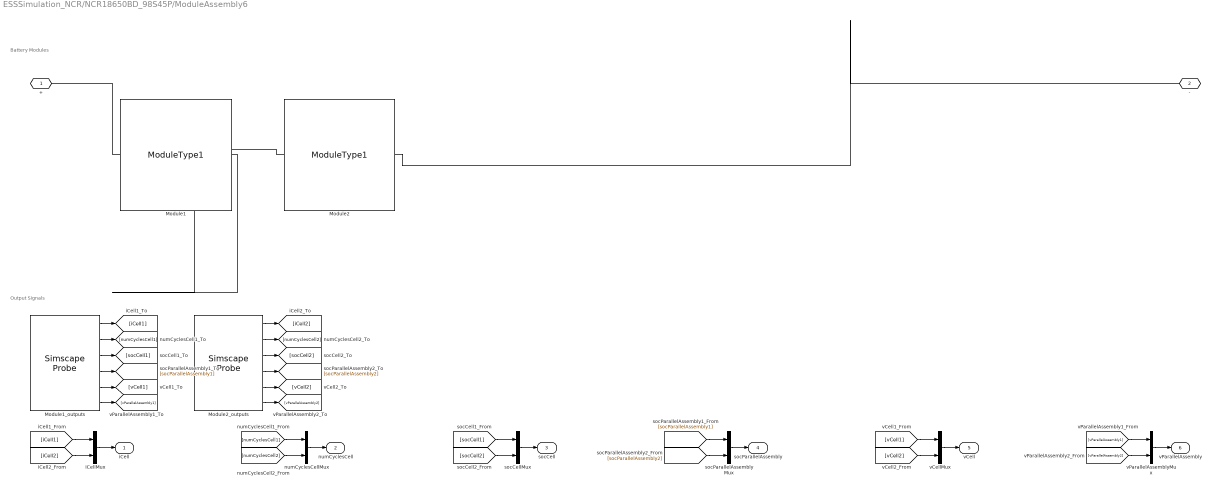
== system ESSSimulation_NCR/NCR18650BD_98S45P/ModuleAssembly6 ==
  note: Battery Modules
  note: Output Signals
  Module1 : NCR18650BD_98S45P_Library_lib/Modules/ModuleType1  SOC_vecCell=[0 0.01 0.02 0.03 0.04 0.05 0.06 0.07 0.08 0.09 0.1 0.11 0.12 0.13 0.14 0.15 0.16 0.17 0.18 0.19 0.2 0.21 0.22 0.23 0.24 0.25 0.26 0.27 0.28 0.29 0.3 0.31 0.32 0.33 0.34 0.35 0.36 0.37 0.38 0.39 0.4 0.41 0.42 0.43 0.44 0.45 0.46 0.47 0.48 0.49 0.5 0.51 0.52 0.53 0.54 0.55 0.56 0.57 0.58 0.59 0.6 0.61 0.62 0.63 0.64 0.65 0.66 0.67 0.68 0.69 0.7 0.71 0.72 0.73 0.74 0.75 0.76 0.77 0.78 0.79 0.8 0.81 0.82 0.83 0.84 0.85 0.86 0.87 0.88 0.89 0.9 0.91 0.92 0.93 0.94 0.95 0.96 0.97 0.98 0.99 1]  V0_vecCell=[2.90003 2.94341 2.98679 3.04987 3.09433 3.12791 3.16031 3.20369 3.23862 3.26689 3.29115 3.31383 3.33202 3.35112 3.36833 3.38413 3.39973 3.41137 3.42149 3.43136 3.44073 3.45027 3.46068 3.47113 3.47814 3.48494 3.49199 3.49905 3.50562 3.51187 3.51861 3.52535 3.53209 3.53818 3.54353 3.54849 3.55353 3.55855 3.56357 3.56831 3.57308 3.57787 3.58264 3.58755 3.5925 3.5985 3.60496 3.61149 3.61805 3.6246 3.63116 3.63855 3.64609 3.65336 3.66064 3.66791 3.67613 3.68522 3.69443 3.70367 3.713 3.72241 3.73154 3.74037 3.7492 3.75786 3.76617 3.77556 3.78485 3.79413 3.8034 3.81149 3.81977 3.82804 3.83631 3.84472 3.85317 3.86155 3.86993 3.87831 3.88686 3.89534 3.90461 3.91454 3.92565 3.93721 3.94924 3.96155 3.97383 3.98598 3.99856 4.01117 4.02361 4.03609 4.04694 4.05695 4.06641 4.07551 4.08514 4.09447 4.10453] V  V_rangeCell=[2.25 Inf] V  R0_vecCell=[0.1741 0.15823 0.14313 0.13285 0.12044 0.10641 0.09605 0.09162 0.08758 0.08349 0.08021 0.07738 0.07487 0.07338 0.07189 0.07117 0.0704 0.06898 0.06755 0.06631 0.06509 0.06388 0.06326 0.06281 0.06182 0.06095 0.06025 0.05955 0.05877 0.05807 0.05761 0.05714 0.05668 0.05611 0.05546 0.0549 0.05439 0.05388 0.05337 0.0528 0.05223 0.05165 0.05106 0.05046 0.04986 0.04945 0.04913 0.04883 0.04854 0.04826 0.04797 0.04782 0.04765 0.0473 0.04695 0.04661 0.04638 0.0463 0.04625 0.04621 0.04624 0.04628 0.04628 0.04623 0.04617 0.04599 0.04573 0.0457 0.04568 0.04565 0.04563 0.04535 0.0451 0.04486 0.04461 0.04446 0.04435 0.04423 0.04411 0.044 0.04372 0.04339 0.04323 0.0432 0.04344 0.04374 0.0441 0.04452 0.04494 0.0454 0.04594 0.0463 0.04649 0.04668 0.04629 0.04541 0.04438 0.04326 0.04154 0.03869 0.03326] Ohm  AHCell=3.153 hr*A  extrapolation_optionCell=simscape.enum.extrapolation.nearest  P=45  S=7  iCell_specify=off  iCell_priority=None  iCell=0 A  iCell_nominal_specify=off  iCell_nominal_value=1  iCell_nominal_unit=A  vCell_specify=off  vCell_priority=None  vCell=0 V  vCell_nominal_specify=off  vCell_nominal_value=1  vCell_nominal_unit=V  socCell_specify=off  socCell_priority=High  socCell=1  socCell_nominal_specify=off  socCell_nominal_value=1  socCell_nominal_unit=1  numCyclesCell_specify=off  numCyclesCell_priority=High  numCyclesCell=0  numCyclesCell_nominal_specify=off  numCyclesCell_nominal_value=1  numCyclesCell_nominal_unit=1  vParallelAssembly_specify=off  vParallelAssembly_priority=None  vParallelAssembly=repmat(0, 7, 1) V  vParallelAssembly_nominal_specify=off  vParallelAssembly_nominal_value=1  vParallelAssembly_nominal_unit=V  socParallelAssembly_specify=off  socParallelAssembly_priority=None  socParallelAssembly=repmat(1, 7, 1)  socParallelAssembly_nominal_specify=off  socParallelAssembly_nominal_value=1  socParallelAssembly_nominal_unit=1
      settings: InternalSimscapePortConfiguration="{\"Bottom\":[{\"id\":\"n\",\"label\":\"-\",\"type\":\"foundation.electrical.electrical\"}],\"Left\":[],\"Right\":[],\"Top\":[{\"id\":\"p\",\"label\":\"+\",\"type\":\"foundation.electrical.electrical\"}]}"
  Module1_outputs : SimscapeProbe  BoundBlock=825  Variables="{\"iCell\":{\"Probing\":\"ON\"},\"numCyclesCell\":{\"Probing\":\"ON\"},\"socCell\":{\"Probing\":\"ON\"},\"socParallelAssembly\":{\"Probing\":\"ON\"},\"vCell\":{\"Probing\":\"ON\"},\"vParallelAssembly\":{\"Probing\":\"ON\"}}"
  Module2 : NCR18650BD_98S45P_Library_lib/Modules/ModuleType1  SOC_vecCell=[0 0.01 0.02 0.03 0.04 0.05 0.06 0.07 0.08 0.09 0.1 0.11 0.12 0.13 0.14 0.15 0.16 0.17 0.18 0.19 0.2 0.21 0.22 0.23 0.24 0.25 0.26 0.27 0.28 0.29 0.3 0.31 0.32 0.33 0.34 0.35 0.36 0.37 0.38 0.39 0.4 0.41 0.42 0.43 0.44 0.45 0.46 0.47 0.48 0.49 0.5 0.51 0.52 0.53 0.54 0.55 0.56 0.57 0.58 0.59 0.6 0.61 0.62 0.63 0.64 0.65 0.66 0.67 0.68 0.69 0.7 0.71 0.72 0.73 0.74 0.75 0.76 0.77 0.78 0.79 0.8 0.81 0.82 0.83 0.84 0.85 0.86 0.87 0.88 0.89 0.9 0.91 0.92 0.93 0.94 0.95 0.96 0.97 0.98 0.99 1]  V0_vecCell=[2.90003 2.94341 2.98679 3.04987 3.09433 3.12791 3.16031 3.20369 3.23862 3.26689 3.29115 3.31383 3.33202 3.35112 3.36833 3.38413 3.39973 3.41137 3.42149 3.43136 3.44073 3.45027 3.46068 3.47113 3.47814 3.48494 3.49199 3.49905 3.50562 3.51187 3.51861 3.52535 3.53209 3.53818 3.54353 3.54849 3.55353 3.55855 3.56357 3.56831 3.57308 3.57787 3.58264 3.58755 3.5925 3.5985 3.60496 3.61149 3.61805 3.6246 3.63116 3.63855 3.64609 3.65336 3.66064 3.66791 3.67613 3.68522 3.69443 3.70367 3.713 3.72241 3.73154 3.74037 3.7492 3.75786 3.76617 3.77556 3.78485 3.79413 3.8034 3.81149 3.81977 3.82804 3.83631 3.84472 3.85317 3.86155 3.86993 3.87831 3.88686 3.89534 3.90461 3.91454 3.92565 3.93721 3.94924 3.96155 3.97383 3.98598 3.99856 4.01117 4.02361 4.03609 4.04694 4.05695 4.06641 4.07551 4.08514 4.09447 4.10453] V  V_rangeCell=[2.25 Inf] V  R0_vecCell=[0.1741 0.15823 0.14313 0.13285 0.12044 0.10641 0.09605 0.09162 0.08758 0.08349 0.08021 0.07738 0.07487 0.07338 0.07189 0.07117 0.0704 0.06898 0.06755 0.06631 0.06509 0.06388 0.06326 0.06281 0.06182 0.06095 0.06025 0.05955 0.05877 0.05807 0.05761 0.05714 0.05668 0.05611 0.05546 0.0549 0.05439 0.05388 0.05337 0.0528 0.05223 0.05165 0.05106 0.05046 0.04986 0.04945 0.04913 0.04883 0.04854 0.04826 0.04797 0.04782 0.04765 0.0473 0.04695 0.04661 0.04638 0.0463 0.04625 0.04621 0.04624 0.04628 0.04628 0.04623 0.04617 0.04599 0.04573 0.0457 0.04568 0.04565 0.04563 0.04535 0.0451 0.04486 0.04461 0.04446 0.04435 0.04423 0.04411 0.044 0.04372 0.04339 0.04323 0.0432 0.04344 0.04374 0.0441 0.04452 0.04494 0.0454 0.04594 0.0463 0.04649 0.04668 0.04629 0.04541 0.04438 0.04326 0.04154 0.03869 0.03326] Ohm  AHCell=3.153 hr*A  extrapolation_optionCell=simscape.enum.extrapolation.nearest  P=45  S=7  iCell_specify=off  iCell_priority=None  iCell=0 A  iCell_nominal_specify=off  iCell_nominal_value=1  iCell_nominal_unit=A  vCell_specify=off  vCell_priority=None  vCell=0 V  vCell_nominal_specify=off  vCell_nominal_value=1  vCell_nominal_unit=V  socCell_specify=off  socCell_priority=High  socCell=1  socCell_nominal_specify=off  socCell_nominal_value=1  socCell_nominal_unit=1  numCyclesCell_specify=off  numCyclesCell_priority=High  numCyclesCell=0  numCyclesCell_nominal_specify=off  numCyclesCell_nominal_value=1  numCyclesCell_nominal_unit=1  vParallelAssembly_specify=off  vParallelAssembly_priority=None  vParallelAssembly=repmat(0, 7, 1) V  vParallelAssembly_nominal_specify=off  vParallelAssembly_nominal_value=1  vParallelAssembly_nominal_unit=V  socParallelAssembly_specify=off  socParallelAssembly_priority=None  socParallelAssembly=repmat(1, 7, 1)  socParallelAssembly_nominal_specify=off  socParallelAssembly_nominal_value=1  socParallelAssembly_nominal_unit=1
      settings: InternalSimscapePortConfiguration="{\"Bottom\":[{\"id\":\"n\",\"label\":\"-\",\"type\":\"foundation.electrical.electrical\"}],\"Left\":[],\"Right\":[],\"Top\":[{\"id\":\"p\",\"label\":\"+\",\"type\":\"foundation.electrical.electrical\"}]}"
  Module2_outputs : SimscapeProbe  BoundBlock=827  Variables="{\"iCell\":{\"Probing\":\"ON\"},\"numCyclesCell\":{\"Probing\":\"ON\"},\"socCell\":{\"Probing\":\"ON\"},\"socParallelAssembly\":{\"Probing\":\"ON\"},\"vCell\":{\"Probing\":\"ON\"},\"vParallelAssembly\":{\"Probing\":\"ON\"}}"
  iCellMux : Mux  Inputs=2
  numCyclesCellMux : Mux  Inputs=2
  socCellMux : Mux  Inputs=2
  socParallelAssemblyMux : Mux  Inputs=2
  vCellMux : Mux  Inputs=2
  vParallelAssemblyMux : Mux  Inputs=2
  + : PMIOPort  Side=Left
  - : PMIOPort  Port=2  Side=Right
  iCell : Outport
  numCyclesCell : Outport  Port=2
  socCell : Outport  Port=3
  socParallelAssembly : Outport  Port=4
  vCell : Outport  Port=5
  vParallelAssembly : Outport  Port=6
  wires:
  Module1_outputs/1 -> [iCell1]
  iCellMux/1 -> iCell/1
  [iCell1] -> iCellMux/1
  Module1_outputs/2 -> [numCyclesCell1]
  numCyclesCellMux/1 -> numCyclesCell/1
  [numCyclesCell1] -> numCyclesCellMux/1
  Module1_outputs/3 -> [socCell1]
  socCellMux/1 -> socCell/1
  [socCell1] -> socCellMux/1
  Module1_outputs/4 -> [socParallelAssembly1]
  socParallelAssemblyMux/1 -> socParallelAssembly/1
  [socParallelAssembly1] -> socParallelAssemblyMux/1
  Module1_outputs/5 -> [vCell1]
  vCellMux/1 -> vCell/1
  [vCell1] -> vCellMux/1
  Module1_outputs/6 -> [vParallelAssembly1]
  vParallelAssemblyMux/1 -> vParallelAssembly/1
  [vParallelAssembly1] -> vParallelAssemblyMux/1
  Module2_outputs/1 -> [iCell2]
  [iCell2] -> iCellMux/2
  Module2_outputs/2 -> [numCyclesCell2]
  [numCyclesCell2] -> numCyclesCellMux/2
  Module2_outputs/3 -> [socCell2]
  [socCell2] -> socCellMux/2
  Module2_outputs/4 -> [socParallelAssembly2]
  [socParallelAssembly2] -> socParallelAssemblyMux/2
  Module2_outputs/5 -> [vCell2]
  [vCell2] -> vCellMux/2
  Module2_outputs/6 -> [vParallelAssembly2]
  [vParallelAssembly2] -> vParallelAssemblyMux/2
  connections:
  Module2/LConn1 -- Module1/RConn1
  Module1/LConn1 -- +/RConn1
  Module2/RConn1 -- -/RConn1

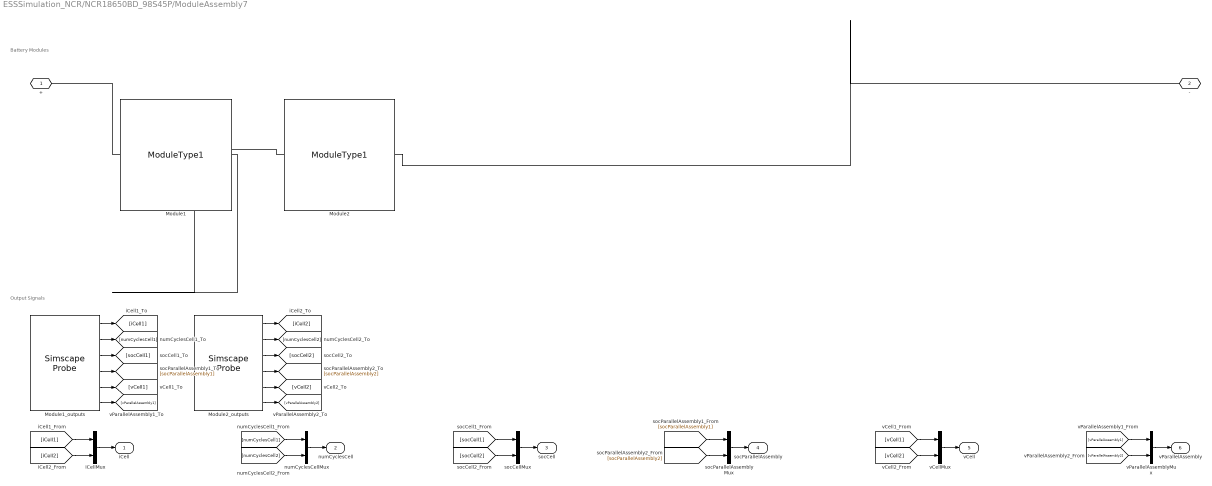
== system ESSSimulation_NCR/NCR18650BD_98S45P/ModuleAssembly7 ==
  note: Battery Modules
  note: Output Signals
  Module1 : NCR18650BD_98S45P_Library_lib/Modules/ModuleType1  SOC_vecCell=[0 0.01 0.02 0.03 0.04 0.05 0.06 0.07 0.08 0.09 0.1 0.11 0.12 0.13 0.14 0.15 0.16 0.17 0.18 0.19 0.2 0.21 0.22 0.23 0.24 0.25 0.26 0.27 0.28 0.29 0.3 0.31 0.32 0.33 0.34 0.35 0.36 0.37 0.38 0.39 0.4 0.41 0.42 0.43 0.44 0.45 0.46 0.47 0.48 0.49 0.5 0.51 0.52 0.53 0.54 0.55 0.56 0.57 0.58 0.59 0.6 0.61 0.62 0.63 0.64 0.65 0.66 0.67 0.68 0.69 0.7 0.71 0.72 0.73 0.74 0.75 0.76 0.77 0.78 0.79 0.8 0.81 0.82 0.83 0.84 0.85 0.86 0.87 0.88 0.89 0.9 0.91 0.92 0.93 0.94 0.95 0.96 0.97 0.98 0.99 1]  V0_vecCell=[2.90003 2.94341 2.98679 3.04987 3.09433 3.12791 3.16031 3.20369 3.23862 3.26689 3.29115 3.31383 3.33202 3.35112 3.36833 3.38413 3.39973 3.41137 3.42149 3.43136 3.44073 3.45027 3.46068 3.47113 3.47814 3.48494 3.49199 3.49905 3.50562 3.51187 3.51861 3.52535 3.53209 3.53818 3.54353 3.54849 3.55353 3.55855 3.56357 3.56831 3.57308 3.57787 3.58264 3.58755 3.5925 3.5985 3.60496 3.61149 3.61805 3.6246 3.63116 3.63855 3.64609 3.65336 3.66064 3.66791 3.67613 3.68522 3.69443 3.70367 3.713 3.72241 3.73154 3.74037 3.7492 3.75786 3.76617 3.77556 3.78485 3.79413 3.8034 3.81149 3.81977 3.82804 3.83631 3.84472 3.85317 3.86155 3.86993 3.87831 3.88686 3.89534 3.90461 3.91454 3.92565 3.93721 3.94924 3.96155 3.97383 3.98598 3.99856 4.01117 4.02361 4.03609 4.04694 4.05695 4.06641 4.07551 4.08514 4.09447 4.10453] V  V_rangeCell=[2.25 Inf] V  R0_vecCell=[0.1741 0.15823 0.14313 0.13285 0.12044 0.10641 0.09605 0.09162 0.08758 0.08349 0.08021 0.07738 0.07487 0.07338 0.07189 0.07117 0.0704 0.06898 0.06755 0.06631 0.06509 0.06388 0.06326 0.06281 0.06182 0.06095 0.06025 0.05955 0.05877 0.05807 0.05761 0.05714 0.05668 0.05611 0.05546 0.0549 0.05439 0.05388 0.05337 0.0528 0.05223 0.05165 0.05106 0.05046 0.04986 0.04945 0.04913 0.04883 0.04854 0.04826 0.04797 0.04782 0.04765 0.0473 0.04695 0.04661 0.04638 0.0463 0.04625 0.04621 0.04624 0.04628 0.04628 0.04623 0.04617 0.04599 0.04573 0.0457 0.04568 0.04565 0.04563 0.04535 0.0451 0.04486 0.04461 0.04446 0.04435 0.04423 0.04411 0.044 0.04372 0.04339 0.04323 0.0432 0.04344 0.04374 0.0441 0.04452 0.04494 0.0454 0.04594 0.0463 0.04649 0.04668 0.04629 0.04541 0.04438 0.04326 0.04154 0.03869 0.03326] Ohm  AHCell=3.153 hr*A  extrapolation_optionCell=simscape.enum.extrapolation.nearest  P=45  S=7  iCell_specify=off  iCell_priority=None  iCell=0 A  iCell_nominal_specify=off  iCell_nominal_value=1  iCell_nominal_unit=A  vCell_specify=off  vCell_priority=None  vCell=0 V  vCell_nominal_specify=off  vCell_nominal_value=1  vCell_nominal_unit=V  socCell_specify=off  socCell_priority=High  socCell=1  socCell_nominal_specify=off  socCell_nominal_value=1  socCell_nominal_unit=1  numCyclesCell_specify=off  numCyclesCell_priority=High  numCyclesCell=0  numCyclesCell_nominal_specify=off  numCyclesCell_nominal_value=1  numCyclesCell_nominal_unit=1  vParallelAssembly_specify=off  vParallelAssembly_priority=None  vParallelAssembly=repmat(0, 7, 1) V  vParallelAssembly_nominal_specify=off  vParallelAssembly_nominal_value=1  vParallelAssembly_nominal_unit=V  socParallelAssembly_specify=off  socParallelAssembly_priority=None  socParallelAssembly=repmat(1, 7, 1)  socParallelAssembly_nominal_specify=off  socParallelAssembly_nominal_value=1  socParallelAssembly_nominal_unit=1
      settings: InternalSimscapePortConfiguration="{\"Bottom\":[{\"id\":\"n\",\"label\":\"-\",\"type\":\"foundation.electrical.electrical\"}],\"Left\":[],\"Right\":[],\"Top\":[{\"id\":\"p\",\"label\":\"+\",\"type\":\"foundation.electrical.electrical\"}]}"
  Module1_outputs : SimscapeProbe  BoundBlock=870  Variables="{\"iCell\":{\"Probing\":\"ON\"},\"numCyclesCell\":{\"Probing\":\"ON\"},\"socCell\":{\"Probing\":\"ON\"},\"socParallelAssembly\":{\"Probing\":\"ON\"},\"vCell\":{\"Probing\":\"ON\"},\"vParallelAssembly\":{\"Probing\":\"ON\"}}"
  Module2 : NCR18650BD_98S45P_Library_lib/Modules/ModuleType1  SOC_vecCell=[0 0.01 0.02 0.03 0.04 0.05 0.06 0.07 0.08 0.09 0.1 0.11 0.12 0.13 0.14 0.15 0.16 0.17 0.18 0.19 0.2 0.21 0.22 0.23 0.24 0.25 0.26 0.27 0.28 0.29 0.3 0.31 0.32 0.33 0.34 0.35 0.36 0.37 0.38 0.39 0.4 0.41 0.42 0.43 0.44 0.45 0.46 0.47 0.48 0.49 0.5 0.51 0.52 0.53 0.54 0.55 0.56 0.57 0.58 0.59 0.6 0.61 0.62 0.63 0.64 0.65 0.66 0.67 0.68 0.69 0.7 0.71 0.72 0.73 0.74 0.75 0.76 0.77 0.78 0.79 0.8 0.81 0.82 0.83 0.84 0.85 0.86 0.87 0.88 0.89 0.9 0.91 0.92 0.93 0.94 0.95 0.96 0.97 0.98 0.99 1]  V0_vecCell=[2.90003 2.94341 2.98679 3.04987 3.09433 3.12791 3.16031 3.20369 3.23862 3.26689 3.29115 3.31383 3.33202 3.35112 3.36833 3.38413 3.39973 3.41137 3.42149 3.43136 3.44073 3.45027 3.46068 3.47113 3.47814 3.48494 3.49199 3.49905 3.50562 3.51187 3.51861 3.52535 3.53209 3.53818 3.54353 3.54849 3.55353 3.55855 3.56357 3.56831 3.57308 3.57787 3.58264 3.58755 3.5925 3.5985 3.60496 3.61149 3.61805 3.6246 3.63116 3.63855 3.64609 3.65336 3.66064 3.66791 3.67613 3.68522 3.69443 3.70367 3.713 3.72241 3.73154 3.74037 3.7492 3.75786 3.76617 3.77556 3.78485 3.79413 3.8034 3.81149 3.81977 3.82804 3.83631 3.84472 3.85317 3.86155 3.86993 3.87831 3.88686 3.89534 3.90461 3.91454 3.92565 3.93721 3.94924 3.96155 3.97383 3.98598 3.99856 4.01117 4.02361 4.03609 4.04694 4.05695 4.06641 4.07551 4.08514 4.09447 4.10453] V  V_rangeCell=[2.25 Inf] V  R0_vecCell=[0.1741 0.15823 0.14313 0.13285 0.12044 0.10641 0.09605 0.09162 0.08758 0.08349 0.08021 0.07738 0.07487 0.07338 0.07189 0.07117 0.0704 0.06898 0.06755 0.06631 0.06509 0.06388 0.06326 0.06281 0.06182 0.06095 0.06025 0.05955 0.05877 0.05807 0.05761 0.05714 0.05668 0.05611 0.05546 0.0549 0.05439 0.05388 0.05337 0.0528 0.05223 0.05165 0.05106 0.05046 0.04986 0.04945 0.04913 0.04883 0.04854 0.04826 0.04797 0.04782 0.04765 0.0473 0.04695 0.04661 0.04638 0.0463 0.04625 0.04621 0.04624 0.04628 0.04628 0.04623 0.04617 0.04599 0.04573 0.0457 0.04568 0.04565 0.04563 0.04535 0.0451 0.04486 0.04461 0.04446 0.04435 0.04423 0.04411 0.044 0.04372 0.04339 0.04323 0.0432 0.04344 0.04374 0.0441 0.04452 0.04494 0.0454 0.04594 0.0463 0.04649 0.04668 0.04629 0.04541 0.04438 0.04326 0.04154 0.03869 0.03326] Ohm  AHCell=3.153 hr*A  extrapolation_optionCell=simscape.enum.extrapolation.nearest  P=45  S=7  iCell_specify=off  iCell_priority=None  iCell=0 A  iCell_nominal_specify=off  iCell_nominal_value=1  iCell_nominal_unit=A  vCell_specify=off  vCell_priority=None  vCell=0 V  vCell_nominal_specify=off  vCell_nominal_value=1  vCell_nominal_unit=V  socCell_specify=off  socCell_priority=High  socCell=1  socCell_nominal_specify=off  socCell_nominal_value=1  socCell_nominal_unit=1  numCyclesCell_specify=off  numCyclesCell_priority=High  numCyclesCell=0  numCyclesCell_nominal_specify=off  numCyclesCell_nominal_value=1  numCyclesCell_nominal_unit=1  vParallelAssembly_specify=off  vParallelAssembly_priority=None  vParallelAssembly=repmat(0, 7, 1) V  vParallelAssembly_nominal_specify=off  vParallelAssembly_nominal_value=1  vParallelAssembly_nominal_unit=V  socParallelAssembly_specify=off  socParallelAssembly_priority=None  socParallelAssembly=repmat(1, 7, 1)  socParallelAssembly_nominal_specify=off  socParallelAssembly_nominal_value=1  socParallelAssembly_nominal_unit=1
      settings: InternalSimscapePortConfiguration="{\"Bottom\":[{\"id\":\"n\",\"label\":\"-\",\"type\":\"foundation.electrical.electrical\"}],\"Left\":[],\"Right\":[],\"Top\":[{\"id\":\"p\",\"label\":\"+\",\"type\":\"foundation.electrical.electrical\"}]}"
  Module2_outputs : SimscapeProbe  BoundBlock=872  Variables="{\"iCell\":{\"Probing\":\"ON\"},\"numCyclesCell\":{\"Probing\":\"ON\"},\"socCell\":{\"Probing\":\"ON\"},\"socParallelAssembly\":{\"Probing\":\"ON\"},\"vCell\":{\"Probing\":\"ON\"},\"vParallelAssembly\":{\"Probing\":\"ON\"}}"
  iCellMux : Mux  Inputs=2
  numCyclesCellMux : Mux  Inputs=2
  socCellMux : Mux  Inputs=2
  socParallelAssemblyMux : Mux  Inputs=2
  vCellMux : Mux  Inputs=2
  vParallelAssemblyMux : Mux  Inputs=2
  + : PMIOPort  Side=Left
  - : PMIOPort  Port=2  Side=Right
  iCell : Outport
  numCyclesCell : Outport  Port=2
  socCell : Outport  Port=3
  socParallelAssembly : Outport  Port=4
  vCell : Outport  Port=5
  vParallelAssembly : Outport  Port=6
  wires:
  Module1_outputs/1 -> [iCell1]
  iCellMux/1 -> iCell/1
  [iCell1] -> iCellMux/1
  Module1_outputs/2 -> [numCyclesCell1]
  numCyclesCellMux/1 -> numCyclesCell/1
  [numCyclesCell1] -> numCyclesCellMux/1
  Module1_outputs/3 -> [socCell1]
  socCellMux/1 -> socCell/1
  [socCell1] -> socCellMux/1
  Module1_outputs/4 -> [socParallelAssembly1]
  socParallelAssemblyMux/1 -> socParallelAssembly/1
  [socParallelAssembly1] -> socParallelAssemblyMux/1
  Module1_outputs/5 -> [vCell1]
  vCellMux/1 -> vCell/1
  [vCell1] -> vCellMux/1
  Module1_outputs/6 -> [vParallelAssembly1]
  vParallelAssemblyMux/1 -> vParallelAssembly/1
  [vParallelAssembly1] -> vParallelAssemblyMux/1
  Module2_outputs/1 -> [iCell2]
  [iCell2] -> iCellMux/2
  Module2_outputs/2 -> [numCyclesCell2]
  [numCyclesCell2] -> numCyclesCellMux/2
  Module2_outputs/3 -> [socCell2]
  [socCell2] -> socCellMux/2
  Module2_outputs/4 -> [socParallelAssembly2]
  [socParallelAssembly2] -> socParallelAssemblyMux/2
  Module2_outputs/5 -> [vCell2]
  [vCell2] -> vCellMux/2
  Module2_outputs/6 -> [vParallelAssembly2]
  [vParallelAssembly2] -> vParallelAssemblyMux/2
  connections:
  Module2/LConn1 -- Module1/RConn1
  Module1/LConn1 -- +/RConn1
  Module2/RConn1 -- -/RConn1
